simulink model "SIL_power_shuffler_sim"  (R2025b)
settings: Solver=VariableStepAuto  StartTime=0.0  StopTime=0.15  MaxStep=1e-4  RelTol=1e-4
PreLoadFcn:
  | P = init_params; CTRL_MODE = 1;
libraries: fl_lib x74, ee_lib x53, nesl_utility x50
(part 1 of 6)
settings Model: SimulationMode=accelerator  Creator=jazsa  LastModifiedBy=jazsa
settings SolverCC: ZeroCrossAlgorithm=Adaptive
settings DataIOCC: SignalLogging=off
settings SFSimCC: SimCustomHeaderCode="#include \"sil_wrappers.h\""
settings SFSimCC: SimUserSources=|
  | firmware/sil/sil_wrappers.c
  | firmware/core/shuffler_ctrl.c
  | firmware/core/shuffler_supervisor.c
  | firmware/core/shuffler_mppt.c
settings SFSimCC: SimUserIncludeDirs=|
  | firmware/sil
  | firmware/core

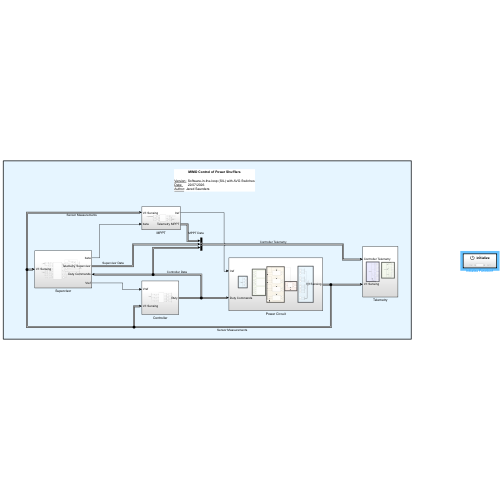
[thumbnail: Simulink's stored preview of the top-level diagram]
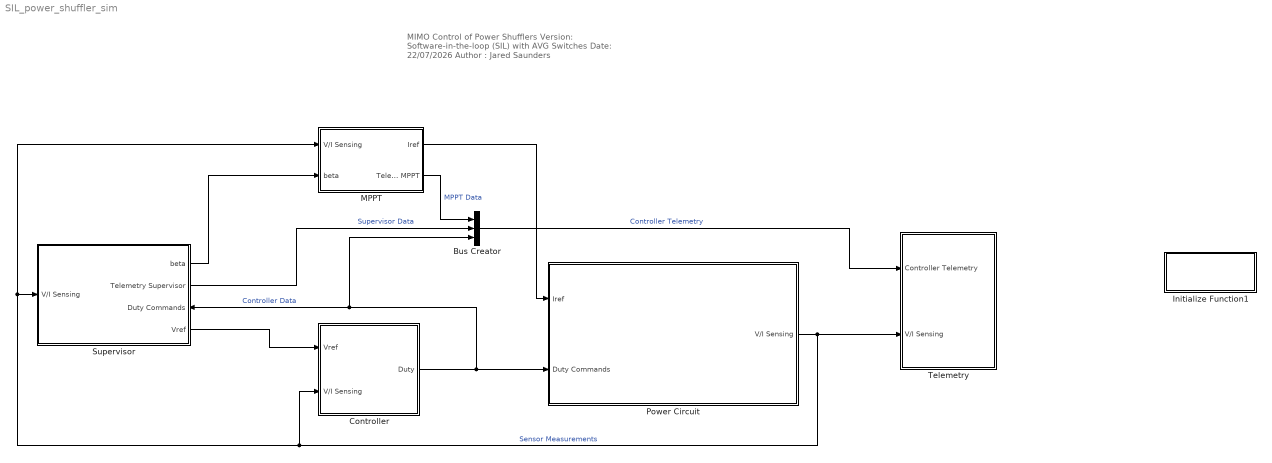
== system SIL_power_shuffler_sim ==
  note: MIMO Control of Power Shufflers
      |
      | Version: Software-in-the-loop (SIL) with AVG Switches
      | Date: 22/07/2026
      | Author : Jared Saunders
  Bus Creator : BusCreator  Inputs=3
  Controller : Subsystem
  Initialize Function1 : Subsystem  TreatAsAtomicUnit=on
  MPPT : Subsystem
  Power Circuit : Subsystem
  Supervisor : Subsystem
      settings: PortSchema="{\"entries\":[{\"content\":{\"sides\":[{\"content\":{\"connectorIds\":[\"In1\"]},\"type\":\"ConnectorPlacement.EquallySpacedRectSide\",\"uuid\":\"551c12cf-3e10-4d97-8eb1-18197da3329a\"},{\"content\":{\"connectorIds\":[\"Out1\",\"Out2\",\"In2\",\"Out3\"],\"side\":\"RIGHT\"},\"type\":\"ConnectorPlacement.EquallySpacedRectSide\",\"uuid\":\"24e69dd1-6804-48d2-9b0c-543d700b19c5\"},{\"content\":{\"side\":\"TOP\"},\"type\":\"ConnectorPlacement.EquallySpacedRectSide\",\"uuid\":\"ec56c192-ffe8-4808-a053-3a704e27c915\"}]},\"type\":\"ConnectorPlacement.EquallySpacedConnector\",\"uuid\":\"0c63dc53-f47f-4434-9688-0d8a13809b3e\"}],\"packageUris\":[\"http://schema.mathworks.com/mf0/Connector/R2020b\"],\"version\":\"1.0\"}"
  Telemetry : Subsystem
  wires:
  MPPT/1(Iref) -> Power Circuit/1(Iref)
  Supervisor/1(beta) -> MPPT/2(beta)
  Power Circuit/1(V/I Sensing) -> Controller/2(V/I Sensing), MPPT/1(V/I Sensing), Supervisor/1(V/I Sensing), Telemetry/2(V/I Sensing)  "Sensor Measurements"
  Supervisor/3(Vref) -> Controller/1(Vref)
  Controller/1(Duty) -> Power Circuit/2(Duty Commands), Bus Creator/3, Supervisor/2(Duty Commands)  "Controller Data"
  MPPT/2(Telemetry MPPT) -> Bus Creator/1  "MPPT Data"
  Supervisor/2(Telemetry Supervisor) -> Bus Creator/2  "Supervisor Data"
  Bus Creator/1 -> Telemetry/1(Controller Telemetry)  "Controller Telemetry"

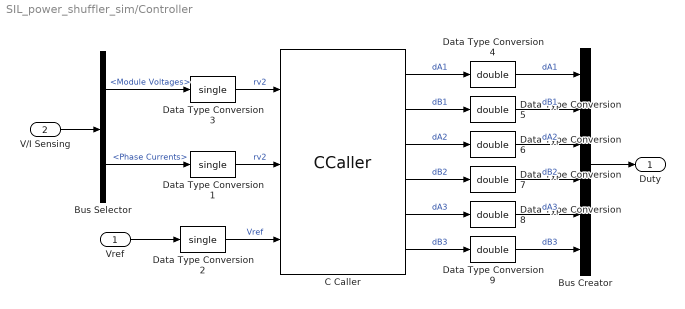
== system SIL_power_shuffler_sim/Controller ==
  Vref : Inport
  V/I Sensing : Inport  Port=2
  Bus Creator : BusCreator  Inputs=6
  Bus Selector : BusSelector  OutputSignals=Module Voltages,Phase Currents
  C Caller : CCaller  FunctionName=sil_ctrl_step  PortSpecificationStruct="%)30     .    & \\   8    (     @         %    \"     D    !     0         %  0 \"0    $    _    07)G3F%M90  4&]R=$YA;64 4V-O<&4     26YD97@     5'EP90      4VEZ90      27-';&]B86P   X    P    !@    @    $          4    (     0    (    !         !   @!630  #@   #     &    \"     0         !0    @    !     @    $         $  \" %9-   .    .     8    (    !          %    \"     $    %     0         0 ...(+4831 chars)"  SampleTime=50e-6
  Data Type Conversion1 : DataTypeConversion  OutDataTypeStr=single  SaturateOnIntegerOverflow=off  RndMeth=Floor
  Data Type Conversion2 : DataTypeConversion  OutDataTypeStr=single  SaturateOnIntegerOverflow=off  RndMeth=Floor
  Data Type Conversion3 : DataTypeConversion  OutDataTypeStr=single  SaturateOnIntegerOverflow=off  RndMeth=Floor
  Data Type Conversion{4..9} (6 alike) : DataTypeConversion  OutDataTypeStr=double  SaturateOnIntegerOverflow=off  RndMeth=Floor
  Duty : Outport
  wires:
  Bus Selector/1 -> Data Type Conversion3/1  "<Module Voltages>"
  C Caller/6 -> Data Type Conversion9/1  "dB3"
  C Caller/5 -> Data Type Conversion8/1  "dA3"
  C Caller/4 -> Data Type Conversion7/1  "dB2"
  C Caller/3 -> Data Type Conversion6/1  "dA2"
  C Caller/2 -> Data Type Conversion5/1  "dB1"
  C Caller/1 -> Data Type Conversion4/1  "dA1"
  Bus Creator/1 -> Duty/1
  V/I Sensing/1 -> Bus Selector/1
  Bus Selector/2 -> Data Type Conversion1/1  "<Phase Currents>"
  Vref/1 -> Data Type Conversion2/1
  Data Type Conversion3/1 -> C Caller/1  "rv2"
  Data Type Conversion1/1 -> C Caller/2  "rv2"
  Data Type Conversion2/1 -> C Caller/3  "Vref"
  Data Type Conversion4/1 -> Bus Creator/1  "dA1"
  Data Type Conversion5/1 -> Bus Creator/2  "dB1"
  Data Type Conversion6/1 -> Bus Creator/3  "dA2"
  Data Type Conversion7/1 -> Bus Creator/4  "dB2"
  Data Type Conversion8/1 -> Bus Creator/5  "dA3"
  Data Type Conversion9/1 -> Bus Creator/6  "dB3"

== system SIL_power_shuffler_sim/Initialize Function1 ==
  C Caller : CCaller  FunctionName=sil_reset_pass  PortSpecificationStruct="%)30     .    N ,   8    (     @         %    \"     (    !     0         %  0 \"0    $    _    07)G3F%M90  4&]R=$YA;64 4V-O<&4     26YD97@     5'EP90      4VEZ90      27-';&]B86P   X    P    !@    @    $          4    (     0    ,    !         !   P!O=70 #@   #     &    \"     0         !0    @    !     P    $         $  # &]U=  .    .     8    (    !          %    \"     $    &     0         0    !@   $]U='!U=   #@   #@    &    \"     8         !0    @    !     0    $         \"0    @               X    X    !@    @    $          4    (     0    8    !         !     &    <VEN9VQE   .    ,     8    (    !          %    \"     $    !     0         0  $ ,0    X    P    !@    @    ) @        4    (     0    $    !          (  0      #@   #     &    \"     0         !0    @    !     0    $         $  ! '4    .    ,     8    (    !          %    \"     $    !     0         0  $ =0    X    X    !@    @    $          4    (     0    4    !         !     %    26YP=70    .    .     8    (    !@         %    \"     $    !     0         )    \"               #@   #@    &    \"     0         !0    @    !    !@    $         $     8   !S:6YG;&4   X    P    !@    @    $          4    (     0    $    !         !   0 Q    #@   #     &    \"     D\"        !0    @    !     0    $          @ !"
  Constant1 : Constant  Value=0
  Data Type Conversion1 : DataTypeConversion  OutDataTypeStr=double  SaturateOnIntegerOverflow=off  RndMeth=Floor
  Data Type Conversion3 : DataTypeConversion  OutDataTypeStr=single  SaturateOnIntegerOverflow=off  RndMeth=Floor
  Event Listener : EventListener  DisableCoverage=on  EventName=reset
  Terminator : Terminator
  wires:
  Constant1/1 -> Data Type Conversion3/1
  Data Type Conversion3/1 -> C Caller/1
  Data Type Conversion1/1 -> Terminator/1
  C Caller/1 -> Data Type Conversion1/1

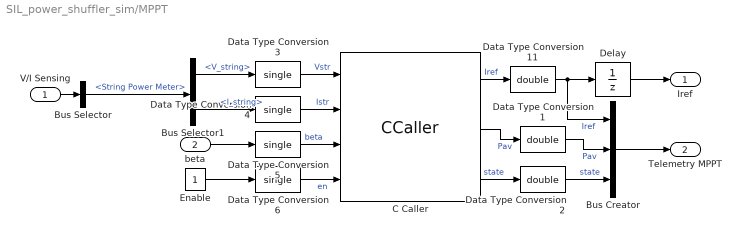
== system SIL_power_shuffler_sim/MPPT ==
  V/I Sensing : Inport
  beta : Inport  Port=2
  Bus Creator : BusCreator  Inputs=3
  Bus Selector : BusSelector  OutputSignals=String Power Meter
  Bus Selector1 : BusSelector  OutputSignals=V_string,I_string
  C Caller : CCaller  FunctionName=sil_mppt_step  PortSpecificationStruct="%)30     .    Z L   8    (     @         %    \"     <    !     0         %  0 \"0    $    _    07)G3F%M90  4&]R=$YA;64 4V-O<&4     26YD97@     5'EP90      4VEZ90      27-';&]B86P   X    P    !@    @    $          4    (     0    0    !         !  ! !6<W1R#@   #     &    \"     0         !0    @    !    !     $         $  $ %9S='(.    .     8    (    !          %    \"     $    %     0         0   ...(+3727 chars)"  SampleTime=1e-3
  Data Type Conversion1 : DataTypeConversion  OutDataTypeStr=double  SaturateOnIntegerOverflow=off  RndMeth=Floor
  Data Type Conversion11 : DataTypeConversion  OutDataTypeStr=double  SaturateOnIntegerOverflow=off  RndMeth=Floor
  Data Type Conversion2 : DataTypeConversion  OutDataTypeStr=double  SaturateOnIntegerOverflow=off  RndMeth=Floor
  Data Type Conversion{3..6} (4 alike) : DataTypeConversion  OutDataTypeStr=single  SaturateOnIntegerOverflow=off  RndMeth=Floor
  Delay : UnitDelay  InitialCondition=12  SampleTime=1e-3  HasFrameUpgradeWarning=on
  Enable : Constant
  Iref : Outport
  Telemetry MPPT : Outport  Port=2
  wires:
  beta/1 -> Data Type Conversion5/1
  Delay/1 -> Iref/1
  C Caller/2 -> Data Type Conversion1/1  "Pav"
  C Caller/3 -> Data Type Conversion2/1  "state"
  C Caller/1 -> Data Type Conversion11/1  "Iref"
  Enable/1 -> Data Type Conversion6/1
  Bus Creator/1 -> Telemetry MPPT/1
  V/I Sensing/1 -> Bus Selector/1
  Bus Selector/1 -> Bus Selector1/1  "<String Power Meter>"
  Bus Selector1/1 -> Data Type Conversion3/1  "<V_string>"
  Bus Selector1/2 -> Data Type Conversion4/1  "<I_string>"
  Data Type Conversion11/1 -> Bus Creator/1, Delay/1  "Iref"
  Data Type Conversion1/1 -> Bus Creator/2  "Pav"
  Data Type Conversion2/1 -> Bus Creator/3  "state"
  Data Type Conversion3/1 -> C Caller/1  "Vstr"
  Data Type Conversion4/1 -> C Caller/2  "Istr"
  Data Type Conversion5/1 -> C Caller/3  "beta"
  Data Type Conversion6/1 -> C Caller/4  "en"

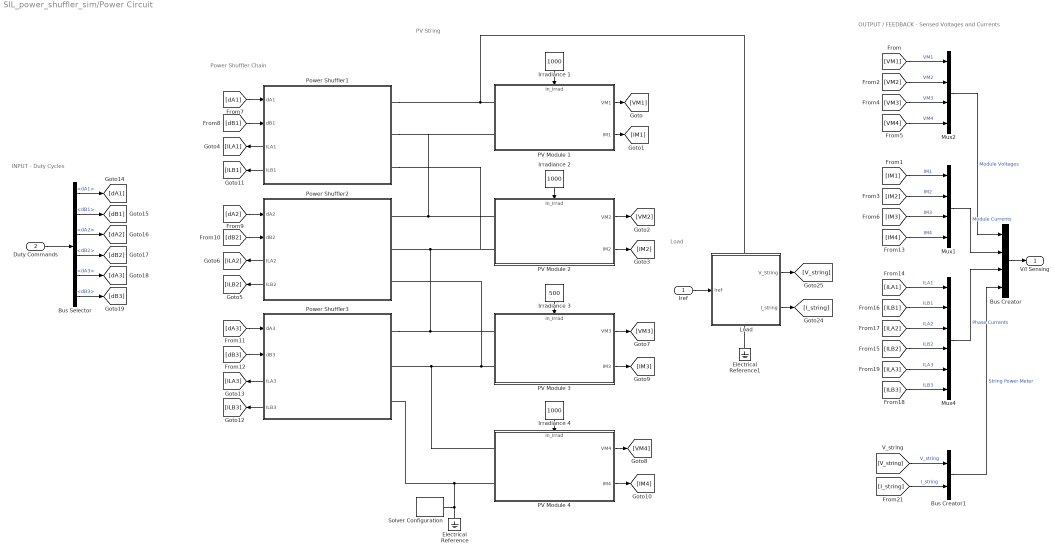
== system SIL_power_shuffler_sim/Power Circuit ==
  note: OUTPUT / FEEDBACK - Sensed Voltages and Currents
  note: Load
  note: PV String
  note: Power Shuffler Chain
  note: INPUT - Duty Cycles
  Iref : Inport
  Duty Commands : Inport  Port=2
  Bus Creator : BusCreator  Inputs=4
  Bus Creator1 : BusCreator  Inputs=2
  Bus Selector : BusSelector  OutputSignals=dA1,dB1,dA2,dB2,dA3,dB3
  Electrical Reference : fl_lib/Electrical/Electrical Elements/Electrical Reference
  Electrical Reference1 : fl_lib/Electrical/Electrical Elements/Electrical Reference
  Irradiance 1 : Constant  Value=1000
  Irradiance 2 : Constant  Value=1000
  Irradiance 3 : Constant  Value=500
  Irradiance 4 : Constant  Value=1000
  Load : Subsystem
      settings: PortSchema="{\"entries\":[{\"content\":{\"sides\":[{\"content\":{\"connectorIds\":[\"LConn1\"]},\"type\":\"ConnectorPlacement.EquallySpacedRectSide\",\"uuid\":\"6f5f716f-38b7-43f9-a9ba-568c6ccf5920\"},{\"content\":{\"connectorIds\":[\"RConn1\"],\"side\":\"RIGHT\"},\"type\":\"ConnectorPlacement.EquallySpacedRectSide\",\"uuid\":\"74a237b1-90a9-413f-978d-7052f4ba1489\"},{\"content\":{\"connectorIds\":[\"In1\"],\"side\":\"TOP\"},\"type\":\"ConnectorPlacement.EquallySpacedRectSide\",\"uuid\":\"e5fcb88f-496e-42e0-91fa-e640406c50d5\"},{\"content\":{\"connectorIds\":[\"Out1\",\"Out2\"],\"side\":\"BOTTOM\"},\"type\":\"ConnectorPlacement.EquallySpacedRectSide\",\"uuid\":\"aed6b45d-7ab9-4ae0-b4e0-d20dd58bb9bf\"}]},\"type\":\"ConnectorPlacement.EquallySpacedConnector\",\"uuid\":\"f6ffe9ce-5007-4054-8c52-fa2588b4e46b\"}],\"packageUris\":[\"http://schema.mathworks.com/mf0/Connector/R2020b\"],\"version\":\"1.0\"}"
  Mux1 : Mux
  Mux2 : Mux
  Mux4 : Mux  Inputs=6
  PV Module 1 : Subsystem
      settings: PortSchema="{\"entries\":[{\"content\":{\"sides\":[{\"content\":{\"connectorIds\":[\"LConn1\",\"LConn2\"]},\"type\":\"ConnectorPlacement.EquallySpacedRectSide\",\"uuid\":\"00bc81be-eb87-4e0d-8cf1-aaf392b111b3\"},{\"content\":{\"connectorIds\":[\"Out1\",\"Out2\"],\"side\":\"RIGHT\"},\"type\":\"ConnectorPlacement.EquallySpacedRectSide\",\"uuid\":\"136cfb59-61d1-4be5-a5a1-62fe670dfe2d\"},{\"content\":{\"connectorIds\":[\"In1\"],\"side\":\"TOP\"},\"type\":\"ConnectorPlacement.EquallySpacedRectSide\",\"uuid\":\"1fa490a3-fddf-446b-98a1-153f2ac018d8\"}]},\"type\":\"ConnectorPlacement.EquallySpacedConnector\",\"uuid\":\"e6ea07bf-3162-47e8-af67-1b2f68d57f24\"}],\"packageUris\":[\"http://schema.mathworks.com/mf0/Connector/R2020b\"],\"version\":\"1.0\"}"
  PV Module 2 : Subsystem
      settings: PortSchema="{\"entries\":[{\"content\":{\"sides\":[{\"content\":{\"connectorIds\":[\"LConn1\",\"LConn2\"]},\"type\":\"ConnectorPlacement.EquallySpacedRectSide\",\"uuid\":\"00bc81be-eb87-4e0d-8cf1-aaf392b111b3\"},{\"content\":{\"connectorIds\":[\"Out1\",\"Out2\"],\"side\":\"RIGHT\"},\"type\":\"ConnectorPlacement.EquallySpacedRectSide\",\"uuid\":\"136cfb59-61d1-4be5-a5a1-62fe670dfe2d\"},{\"content\":{\"connectorIds\":[\"In1\"],\"side\":\"TOP\"},\"type\":\"ConnectorPlacement.EquallySpacedRectSide\",\"uuid\":\"1fa490a3-fddf-446b-98a1-153f2ac018d8\"}]},\"type\":\"ConnectorPlacement.EquallySpacedConnector\",\"uuid\":\"e6ea07bf-3162-47e8-af67-1b2f68d57f24\"}],\"packageUris\":[\"http://schema.mathworks.com/mf0/Connector/R2020b\"],\"version\":\"1.0\"}"
  PV Module 3 : Subsystem
      settings: PortSchema="{\"entries\":[{\"content\":{\"sides\":[{\"content\":{\"connectorIds\":[\"LConn1\",\"LConn2\"]},\"type\":\"ConnectorPlacement.EquallySpacedRectSide\",\"uuid\":\"00bc81be-eb87-4e0d-8cf1-aaf392b111b3\"},{\"content\":{\"connectorIds\":[\"Out1\",\"Out2\"],\"side\":\"RIGHT\"},\"type\":\"ConnectorPlacement.EquallySpacedRectSide\",\"uuid\":\"136cfb59-61d1-4be5-a5a1-62fe670dfe2d\"},{\"content\":{\"connectorIds\":[\"In1\"],\"side\":\"TOP\"},\"type\":\"ConnectorPlacement.EquallySpacedRectSide\",\"uuid\":\"1fa490a3-fddf-446b-98a1-153f2ac018d8\"}]},\"type\":\"ConnectorPlacement.EquallySpacedConnector\",\"uuid\":\"e6ea07bf-3162-47e8-af67-1b2f68d57f24\"}],\"packageUris\":[\"http://schema.mathworks.com/mf0/Connector/R2020b\"],\"version\":\"1.0\"}"
  PV Module 4 : Subsystem
      settings: PortSchema="{\"entries\":[{\"content\":{\"sides\":[{\"content\":{\"connectorIds\":[\"LConn1\",\"LConn2\"]},\"type\":\"ConnectorPlacement.EquallySpacedRectSide\",\"uuid\":\"00bc81be-eb87-4e0d-8cf1-aaf392b111b3\"},{\"content\":{\"connectorIds\":[\"Out1\",\"Out2\"],\"side\":\"RIGHT\"},\"type\":\"ConnectorPlacement.EquallySpacedRectSide\",\"uuid\":\"136cfb59-61d1-4be5-a5a1-62fe670dfe2d\"},{\"content\":{\"connectorIds\":[\"In1\"],\"side\":\"TOP\"},\"type\":\"ConnectorPlacement.EquallySpacedRectSide\",\"uuid\":\"1fa490a3-fddf-446b-98a1-153f2ac018d8\"}]},\"type\":\"ConnectorPlacement.EquallySpacedConnector\",\"uuid\":\"e6ea07bf-3162-47e8-af67-1b2f68d57f24\"}],\"packageUris\":[\"http://schema.mathworks.com/mf0/Connector/R2020b\"],\"version\":\"1.0\"}"
  Power Shuffler1 : Subsystem
      settings: PortSchema="{\"entries\":[{\"content\":{\"sides\":[{\"content\":{\"connectorIds\":[\"LConn1\",\"LConn2\",\"LConn3\"]},\"type\":\"ConnectorPlacement.EquallySpacedRectSide\",\"uuid\":\"00177d11-8382-42fd-b27c-fc09158175e4\"},{\"content\":{\"connectorIds\":[\"In1\",\"In2\",\"Out1\",\"Out2\"],\"side\":\"RIGHT\"},\"type\":\"ConnectorPlacement.EquallySpacedRectSide\",\"uuid\":\"90a306f0-da10-41e1-a725-cfb753adc00c\"},{\"content\":{\"side\":\"TOP\"},\"type\":\"ConnectorPlacement.EquallySpacedRectSide\",\"uuid\":\"612e5683-3ee7-4398-9a5a-0cbdc6c6e41b\"}]},\"type\":\"ConnectorPlacement.EquallySpacedConnector\",\"uuid\":\"1790a0ac-9047-4198-9955-1e7cd181ed81\"}],\"packageUris\":[\"http://schema.mathworks.com/mf0/Connector/R2020b\"],\"version\":\"1.0\"}"
  Power Shuffler2 : Subsystem
      settings: PortSchema="{\"entries\":[{\"content\":{\"sides\":[{\"content\":{\"connectorIds\":[\"LConn1\",\"LConn2\",\"LConn3\"]},\"type\":\"ConnectorPlacement.EquallySpacedRectSide\",\"uuid\":\"00177d11-8382-42fd-b27c-fc09158175e4\"},{\"content\":{\"connectorIds\":[\"In1\",\"In2\",\"Out1\",\"Out2\"],\"side\":\"RIGHT\"},\"type\":\"ConnectorPlacement.EquallySpacedRectSide\",\"uuid\":\"90a306f0-da10-41e1-a725-cfb753adc00c\"},{\"content\":{\"side\":\"TOP\"},\"type\":\"ConnectorPlacement.EquallySpacedRectSide\",\"uuid\":\"612e5683-3ee7-4398-9a5a-0cbdc6c6e41b\"}]},\"type\":\"ConnectorPlacement.EquallySpacedConnector\",\"uuid\":\"1790a0ac-9047-4198-9955-1e7cd181ed81\"}],\"packageUris\":[\"http://schema.mathworks.com/mf0/Connector/R2020b\"],\"version\":\"1.0\"}"
  Power Shuffler3 : Subsystem
      settings: PortSchema="{\"entries\":[{\"content\":{\"sides\":[{\"content\":{\"connectorIds\":[\"LConn1\",\"LConn2\",\"LConn3\"]},\"type\":\"ConnectorPlacement.EquallySpacedRectSide\",\"uuid\":\"00177d11-8382-42fd-b27c-fc09158175e4\"},{\"content\":{\"connectorIds\":[\"In1\",\"In2\",\"Out1\",\"Out2\"],\"side\":\"RIGHT\"},\"type\":\"ConnectorPlacement.EquallySpacedRectSide\",\"uuid\":\"90a306f0-da10-41e1-a725-cfb753adc00c\"},{\"content\":{\"side\":\"TOP\"},\"type\":\"ConnectorPlacement.EquallySpacedRectSide\",\"uuid\":\"612e5683-3ee7-4398-9a5a-0cbdc6c6e41b\"}]},\"type\":\"ConnectorPlacement.EquallySpacedConnector\",\"uuid\":\"1790a0ac-9047-4198-9955-1e7cd181ed81\"}],\"packageUris\":[\"http://schema.mathworks.com/mf0/Connector/R2020b\"],\"version\":\"1.0\"}"
  Solver Configuration : nesl_utility/Solver Configuration  PhysicalDomain=network_engine_domain  SubClassName=solver  LeftPortType=input  RightPortType=generic  Tones=[]  Harmonics=[]  SimulateNoise=off  Profile=off  UseLocalSampling=off  EnableSwitchedLinearOptims=on  FrequencyDomain=off  UseCCode=off  RelTol=0.001  AbsTol=0.001  MinStep=1e-09  ToWorkspace=off  RevertToSquareIcSolve=off  NumHomotopyIterations=100  PhasorMode=off  PhasorModeNumHarmonics=1  ConsistencySolver=NEWTON_XTOL_AFTER_FTOL  IndexReductionMethod=DerivativeReplacement  DoDC=off  ResidualTolerance=1e-09  ConsistencyTolSource=GLOBAL  ConsistencyAbsTol=0.001  ConsistencyRelTol=0.001  ConsistencyTolFactor=0.001  UseLocalSolver=on  LocalSolverChoice=NE_BACKWARD_EULER_ADVANCER  ResolveIndetEquations=on  FunctionEvalNumThread=1  LocalSolverSampleTime=1e-7  DoFixedCost=off  MaxNonlinIter=3  MaxModeIter=2  ComputeImpulses=off  ImpulseIterations=2  LinearAlgebra=auto  LinearAlgebraNumThread=0  EquationFormulation=NE_TIME_EF  DelaysMemoryBudget=1024  AutomaticFiltering=on  FilteringTimeConstant=0.001  PartitionStorageMethod=AS_NEEDED  PartitionMemoryBudget=1024  PartitionMethod=ROBUST  MultibodyUseLocalSolver=off  MultibodyLocalSolverChoice=ODE1  MultibodyLocalSolverSampleTime=0.001
  V/I Sensing : Outport
  wires:
  Iref/1 -> Load/1(Iref)
  Load/2(V_String) -> [V_string]
  PV Module 1/1(VM1) -> [VM1]
  Load/1(I_string) -> [I_string]
  Irradiance 3/1 -> PV Module 3/1(In_Irrad)
  Irradiance 4/1 -> PV Module 4/1(In_Irrad)
  Irradiance 2/1 -> PV Module 2/1(In_Irrad)
  Irradiance 1/1 -> PV Module 1/1(In_Irrad)
  Mux2/1 -> Bus Creator/1  "Module Voltages"
  Mux1/1 -> Bus Creator/2  "Module Currents"
  [VM1] -> Mux2/1  "VM1"
  PV Module 1/2(IM1) -> [IM1]
  [IM1] -> Mux1/1  "IM1"
  PV Module 2/1(VM2) -> [VM2]
  [VM2] -> Mux2/2  "VM2"
  PV Module 2/2(IM2) -> [IM2]
  [VM3] -> Mux2/3  "VM3"
  [IM2] -> Mux1/2  "IM2"
  PV Module 3/1(VM3) -> [VM3]
  PV Module 4/1(VM4) -> [VM4]
  [VM4] -> Mux2/4  "VM4"
  PV Module 3/2(IM3) -> [IM3]
  [IM3] -> Mux1/3  "IM3"
  PV Module 4/2(IM4) -> [IM4]
  [IM4] -> Mux1/4  "IM4"
  Power Shuffler1/1(ILA1) -> [ILA1]
  Power Shuffler1/2(ILB1) -> [ILB1]
  Power Shuffler2/2(ILB2) -> [ILB2]
  Power Shuffler2/1(ILA2) -> [ILA2]
  Power Shuffler3/2(ILB3) -> [ILB3]
  Power Shuffler3/1(ILA3) -> [ILA3]
  [ILB3] -> Mux4/6  "ILB3"
  [ILA3] -> Mux4/5  "ILA3"
  [ILA1] -> Mux4/1  "ILA1"
  [ILA2] -> Mux4/3  "ILA2"
  [ILB1] -> Mux4/2  "ILB1"
  [ILB2] -> Mux4/4  "ILB2"
  Mux4/1 -> Bus Creator/3  "Phase Currents"
  [dA1] -> Power Shuffler1/1(dA1)
  Duty Commands/1 -> Bus Selector/1
  Bus Selector/1 -> [dA1]  "<dA1>"
  Bus Selector/2 -> [dB1]  "<dB1>"
  [dB1] -> Power Shuffler1/2(dB1)
  [dB2] -> Power Shuffler2/2(dB2)
  [dA2] -> Power Shuffler2/1(dA2)
  [dA3] -> Power Shuffler3/1(dA3)
  [dB3] -> Power Shuffler3/2(dB3)
  Bus Selector/4 -> [dB2]  "<dB2>"
  Bus Selector/3 -> [dA2]  "<dA2>"
  Bus Selector/6 -> [dB3]  "<dB3>"
  Bus Selector/5 -> [dA3]  "<dA3>"
  [V_string] -> Bus Creator1/1  "V_string"
  [I_string] -> Bus Creator1/2  "I_string"
  Bus Creator/1 -> V/I Sensing/1
  Bus Creator1/1 -> Bus Creator/4  "String Power Meter"
  connections:
  PV Module 1/LConn2 -- Power Shuffler1/LConn2 -- PV Module 2/LConn1 -- Power Shuffler2/LConn1
  PV Module 1/LConn1 -- Load/RConn1 -- Power Shuffler1/LConn1
  PV Module 3/LConn1 -- PV Module 2/LConn2 -- Power Shuffler1/LConn3 -- Power Shuffler2/LConn2 -- Power Shuffler3/LConn1
  Solver Configuration/RConn1 -- Power Shuffler3/LConn3 -- PV Module 4/LConn2 -- Electrical Reference/LConn1
  PV Module 3/LConn2 -- PV Module 4/LConn1 -- Power Shuffler3/LConn2 -- Power Shuffler2/LConn3
  Electrical Reference1/LConn1 -- Load/LConn1

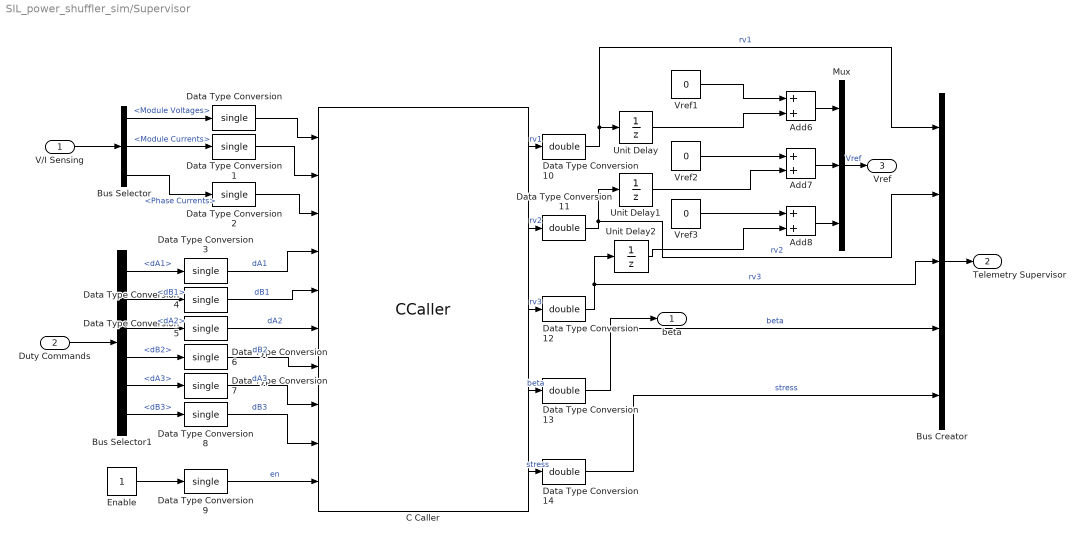
== system SIL_power_shuffler_sim/Supervisor ==
  V/I Sensing : Inport
  Duty Commands : Inport  Port=2
  Add6 : Sum
  Add7 : Sum
  Add8 : Sum
  Bus Creator : BusCreator  Inputs=5
  Bus Selector : BusSelector  OutputSignals=Module Voltages,Module Currents,Phase Currents
  Bus Selector1 : BusSelector  OutputSignals=dA1,dB1,dA2,dB2,dA3,dB3
  C Caller : CCaller  FunctionName=sil_supervisor_step  PortSpecificationStruct="%)30     .    Z!@   8    (     @         %    \"     \\    !     0         %  0 \"0    $    _    07)G3F%M90  4&]R=$YA;64 4V-O<&4     26YD97@     5'EP90      4VEZ90      27-';&]B86P   X    P    !@    @    $          4    (     0    (    !         !   @!630  #@   #     &    \"     0         !0    @    !     @    $         $  \" %9-   .    .     8    (    !          %    \"     $    %     0         0 ...(+8221 chars)"  SampleTime=1e-3
  Data Type Conversion{,1..9} (10 alike) : DataTypeConversion  OutDataTypeStr=single  SaturateOnIntegerOverflow=off  RndMeth=Floor
  Data Type Conversion{10..14} (5 alike) : DataTypeConversion  OutDataTypeStr=double  SaturateOnIntegerOverflow=off  RndMeth=Floor
  Enable : Constant
  Mux : Mux  Inputs=3
  Unit Delay : UnitDelay  SampleTime=1e-3  HasFrameUpgradeWarning=on
  Unit Delay1 : UnitDelay  SampleTime=1e-3  HasFrameUpgradeWarning=on
  Unit Delay2 : UnitDelay  SampleTime=1e-3  HasFrameUpgradeWarning=on
  Vref1 : Constant  Value=0
  Vref2 : Constant  Value=0
  Vref3 : Constant  Value=0
  beta : Outport
  Telemetry Supervisor : Outport  Port=2
  Vref : Outport  Port=3
  wires:
  Data Type Conversion12/1 -> Unit Delay2/1, Bus Creator/3  "rv3"
  Data Type Conversion10/1 -> Bus Creator/1, Unit Delay/1  "rv1"
  Data Type Conversion13/1 -> beta/1, Bus Creator/4  "beta"
  Data Type Conversion14/1 -> Bus Creator/5  "stress"
  Enable/1 -> Data Type Conversion9/1
  Data Type Conversion11/1 -> Unit Delay1/1, Bus Creator/2  "rv2"
  Mux/1 -> Vref/1  "Vref"
  Add8/1 -> Mux/3
  Add7/1 -> Mux/2
  Unit Delay1/1 -> Add7/2
  Unit Delay2/1 -> Add8/2
  Vref2/1 -> Add7/1
  Add6/1 -> Mux/1
  Unit Delay/1 -> Add6/2
  Vref1/1 -> Add6/1
  Vref3/1 -> Add8/1
  Bus Creator/1 -> Telemetry Supervisor/1
  V/I Sensing/1 -> Bus Selector/1
  Bus Selector/1 -> Data Type Conversion/1  "<Module Voltages>"
  Bus Selector/2 -> Data Type Conversion1/1  "<Module Currents>"
  Bus Selector/3 -> Data Type Conversion2/1  "<Phase Currents>"
  Bus Selector1/1 -> Data Type Conversion3/1  "<dA1>"
  Bus Selector1/6 -> Data Type Conversion8/1  "<dB3>"
  Bus Selector1/5 -> Data Type Conversion7/1  "<dA3>"
  Bus Selector1/4 -> Data Type Conversion6/1  "<dB2>"
  Bus Selector1/2 -> Data Type Conversion4/1  "<dB1>"
  Bus Selector1/3 -> Data Type Conversion5/1  "<dA2>"
  Duty Commands/1 -> Bus Selector1/1
  Data Type Conversion/1 -> C Caller/1
  Data Type Conversion1/1 -> C Caller/2
  Data Type Conversion2/1 -> C Caller/3
  Data Type Conversion3/1 -> C Caller/4  "dA1"
  Data Type Conversion4/1 -> C Caller/5  "dB1"
  Data Type Conversion5/1 -> C Caller/6  "dA2"
  Data Type Conversion6/1 -> C Caller/7  "dB2"
  Data Type Conversion7/1 -> C Caller/8  "dA3"
  Data Type Conversion8/1 -> C Caller/9  "dB3"
  Data Type Conversion9/1 -> C Caller/10  "en"
  C Caller/1 -> Data Type Conversion10/1  "rv1"
  C Caller/2 -> Data Type Conversion11/1  "rv2"
  C Caller/3 -> Data Type Conversion12/1  "rv3"
  C Caller/4 -> Data Type Conversion13/1  "beta"
  C Caller/5 -> Data Type Conversion14/1  "stress"

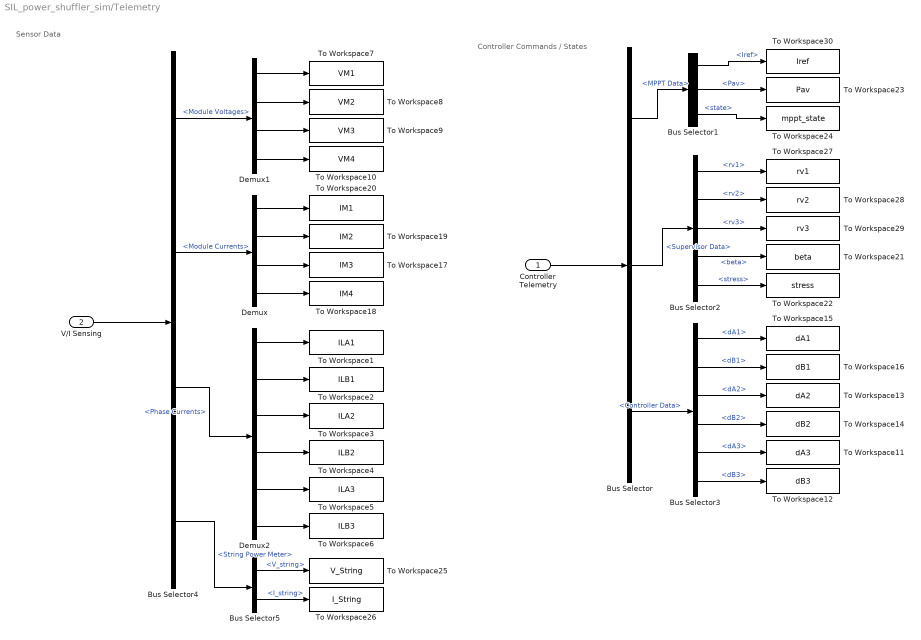
== system SIL_power_shuffler_sim/Telemetry ==
  note: Controller Commands / States
  note: Sensor Data
  Controller Telemetry : Inport
  V/I Sensing : Inport  Port=2
  Bus Selector : BusSelector  OutputSignals=MPPT Data,Supervisor Data,Controller Data
  Bus Selector1 : BusSelector  OutputSignals=Iref,Pav,state
  Bus Selector2 : BusSelector  OutputSignals=rv1,rv2,rv3,beta,stress
  Bus Selector3 : BusSelector  OutputSignals=dA1,dB1,dA2,dB2,dA3,dB3
  Bus Selector4 : BusSelector  OutputSignals=Module Voltages,Module Currents,Phase Currents,String Power Meter
  Bus Selector5 : BusSelector  OutputSignals=V_string,I_string
  Demux : Demux
  Demux1 : Demux
  Demux2 : Demux  Outputs=6
  To Workspace1 : ToWorkspace  VariableName=ILA1  SaveFormat=Timeseries  SampleTime=-1
  To Workspace10 : ToWorkspace  VariableName=VM4  SaveFormat=Timeseries  SampleTime=-1
  To Workspace11 : ToWorkspace  VariableName=dA3  SaveFormat=Timeseries  SampleTime=-1
  To Workspace12 : ToWorkspace  VariableName=dB3  SaveFormat=Timeseries  SampleTime=-1
  To Workspace13 : ToWorkspace  VariableName=dA2  SaveFormat=Timeseries  SampleTime=-1
  To Workspace14 : ToWorkspace  VariableName=dB2  SaveFormat=Timeseries  SampleTime=-1
  To Workspace15 : ToWorkspace  VariableName=dA1  SaveFormat=Timeseries  SampleTime=-1
  To Workspace16 : ToWorkspace  VariableName=dB1  SaveFormat=Timeseries  SampleTime=-1
  To Workspace17 : ToWorkspace  VariableName=IM3  SaveFormat=Timeseries  SampleTime=-1
  To Workspace18 : ToWorkspace  VariableName=IM4  SaveFormat=Timeseries  SampleTime=-1
  To Workspace19 : ToWorkspace  VariableName=IM2  SaveFormat=Timeseries  SampleTime=-1
  To Workspace2 : ToWorkspace  VariableName=ILB1  SaveFormat=Timeseries  SampleTime=-1
  To Workspace20 : ToWorkspace  VariableName=IM1  SaveFormat=Timeseries  SampleTime=-1
  To Workspace21 : ToWorkspace  VariableName=beta  SaveFormat=Timeseries  SampleTime=-1
  To Workspace22 : ToWorkspace  VariableName=stress  SaveFormat=Timeseries  SampleTime=-1
  To Workspace23 : ToWorkspace  VariableName=Pav  SaveFormat=Timeseries  SampleTime=-1
  To Workspace24 : ToWorkspace  VariableName=mppt_state  SaveFormat=Timeseries  SampleTime=-1
  To Workspace25 : ToWorkspace  VariableName=V_String  SaveFormat=Timeseries  SampleTime=-1
  To Workspace26 : ToWorkspace  VariableName=I_String  SaveFormat=Timeseries  SampleTime=-1
  To Workspace27 : ToWorkspace  VariableName=rv1  SaveFormat=Timeseries  SampleTime=-1
  To Workspace28 : ToWorkspace  VariableName=rv2  SaveFormat=Timeseries  SampleTime=-1
  To Workspace29 : ToWorkspace  VariableName=rv3  SaveFormat=Timeseries  SampleTime=-1
  To Workspace3 : ToWorkspace  VariableName=ILA2  SaveFormat=Timeseries  SampleTime=-1
  To Workspace30 : ToWorkspace  VariableName=Iref  SaveFormat=Timeseries  SampleTime=-1
  To Workspace4 : ToWorkspace  VariableName=ILB2  SaveFormat=Timeseries  SampleTime=-1
  To Workspace5 : ToWorkspace  VariableName=ILA3  SaveFormat=Timeseries  SampleTime=-1
  To Workspace6 : ToWorkspace  VariableName=ILB3  SaveFormat=Timeseries  SampleTime=-1
  To Workspace7 : ToWorkspace  VariableName=VM1  SaveFormat=Timeseries  SampleTime=-1
  To Workspace8 : ToWorkspace  VariableName=VM2  SaveFormat=Timeseries  SampleTime=-1
  To Workspace9 : ToWorkspace  VariableName=VM3  SaveFormat=Timeseries  SampleTime=-1
  wires:
  V/I Sensing/1 -> Bus Selector4/1
  Controller Telemetry/1 -> Bus Selector/1
  Bus Selector1/2 -> To Workspace23/1  "<Pav>"
  Bus Selector/1 -> Bus Selector1/1  "<MPPT Data>"
  Bus Selector1/3 -> To Workspace24/1  "<state>"
  Bus Selector/2 -> Bus Selector2/1  "<Supervisor Data>"
  Bus Selector2/4 -> To Workspace21/1  "<beta>"
  Bus Selector2/5 -> To Workspace22/1  "<stress>"
  Bus Selector/3 -> Bus Selector3/1  "<Controller Data>"
  Bus Selector3/2 -> To Workspace16/1  "<dB1>"
  Bus Selector3/6 -> To Workspace12/1  "<dB3>"
  Bus Selector3/5 -> To Workspace11/1  "<dA3>"
  Bus Selector3/4 -> To Workspace14/1  "<dB2>"
  Bus Selector3/3 -> To Workspace13/1  "<dA2>"
  Bus Selector3/1 -> To Workspace15/1  "<dA1>"
  Bus Selector4/2 -> Demux/1  "<Module Currents>"
  Demux/1 -> To Workspace20/1
  Demux/2 -> To Workspace19/1
  Demux/3 -> To Workspace17/1
  Demux/4 -> To Workspace18/1
  Bus Selector4/1 -> Demux1/1  "<Module Voltages>"
  Demux1/1 -> To Workspace7/1
  Demux1/2 -> To Workspace8/1
  Demux1/3 -> To Workspace9/1
  Demux1/4 -> To Workspace10/1
  Bus Selector4/3 -> Demux2/1  "<Phase Currents>"
  Demux2/1 -> To Workspace1/1
  Demux2/2 -> To Workspace2/1
  Demux2/3 -> To Workspace3/1
  Demux2/4 -> To Workspace4/1
  Demux2/5 -> To Workspace5/1
  Demux2/6 -> To Workspace6/1
  Bus Selector4/4 -> Bus Selector5/1  "<String Power Meter>"
  Bus Selector5/1 -> To Workspace25/1  "<V_string>"
  Bus Selector5/2 -> To Workspace26/1  "<I_string>"
  Bus Selector2/2 -> To Workspace28/1  "<rv2>"
  Bus Selector2/1 -> To Workspace27/1  "<rv1>"
  Bus Selector2/3 -> To Workspace29/1  "<rv3>"
  Bus Selector1/1 -> To Workspace30/1  "<Iref>"

== system SIL_power_shuffler_sim/Power Circuit/Load ==
  Iref : Inport
  Controlled Current Source : fl_lib/Electrical/Electrical Sources/Controlled Current Source
  Current Sensor : fl_lib/Electrical/Electrical Sensors/Current Sensor
  PS-Simulink Converter : nesl_utility/PS-Simulink Converter  PhysicalDomain=network_engine_domain  SubClassName=ps_output  LeftPortType=input  RightPortType=output  PseudoPeriodic=off  Frequencies=[]  VectorFormat=inherit  Unit=inherit  AffineConversion=off
  PS-Simulink Converter1 : nesl_utility/PS-Simulink Converter  PhysicalDomain=network_engine_domain  SubClassName=ps_output  LeftPortType=input  RightPortType=output  PseudoPeriodic=off  Frequencies=[]  VectorFormat=inherit  Unit=inherit  AffineConversion=off
  Simulink-PS Converter : nesl_utility/Simulink-PS Converter  PhysicalDomain=network_engine_domain  SubClassName=ps_input  LeftPortType=input  RightPortType=output  PseudoPeriodic=off  Frequencies=[]  NoiseDistribution=none  NoiseParameters=[]  Unit=1  AffineConversion=off  FilteringAndDerivatives=provide  SimscapeFilterOrder=1  InputFilterTimeConstant=0.001  UdotUserProvided=0
  Voltage Sensor : fl_lib/Electrical/Electrical Sensors/Voltage Sensor
  -ve Terminal : PMIOPort  Side=Left
  +Ve Terminal : PMIOPort  Port=2  Side=Right
  I_string : Outport
  V_String : Outport  Port=2
  wires:
  PS-Simulink Converter/1 -> V_String/1
  PS-Simulink Converter1/1 -> I_string/1
  Iref/1 -> Simulink-PS Converter/1
  connections:
  Voltage Sensor/RConn1 -- PS-Simulink Converter/LConn1
  +Ve Terminal/RConn1 -- Controlled Current Source/RConn2 -- Voltage Sensor/LConn1
  Voltage Sensor/RConn2 -- Current Sensor/RConn2 -- -ve Terminal/RConn1
  Current Sensor/RConn1 -- PS-Simulink Converter1/LConn1
  Controlled Current Source/LConn1 -- Current Sensor/LConn1
  Simulink-PS Converter/RConn1 -- Controlled Current Source/RConn1
